simulink model "SensorlessHandoverTest"  (R2026b)
settings: Solver=FixedStepDiscrete  StopTime=handoverTestCfg.Duration  FixedStep=handoverCfg.Ts
PostLoadFcn:
  | addpath(fullfile(fileparts(get_param(bdroot,'FileName')),'..','build_process'));initialize_handover_test(bdroot);
model workspace (MAT data in the model file):
  handoverCfg.Ts = 5e-05
  handoverCfg.MinOmega = 100
  handoverCfg.MaxSpeedGap = 80
  handoverCfg.MaxPhaseGap = 0.9
  handoverCfg.MaxResidual = 1.5
  handoverCfg.CaptureTime = 0.01
  handoverCfg.BlendTime = 0.1
  handoverCfg.LossTime = 0.001
  handoverCfg.MaxPhaseInnovation = 0.15
  handoverCfg.AllowFlying = 1
  handoverCfg.Samples = [200; 2000; 20]
  handoverCfg.Vector = [5e-05; 100; 80; 0.9; 1.5; 200; 2000; 20; 0.15; 1]
  handoverCfg.State0 = [0; 0; 0; 0; 0; 0; 0; 0; 0]
  handoverTestCfg.Duration = 0.35
  handoverTestCfg.ElectricalSpeed = 200
  handoverTestCfg.InitialAngle = 0
  handoverTestCfg.StartupAngleOffset = 0.4
  handoverTestCfg.Ready = 1
  handoverTestCfg.StartupMode = 4
  handoverTestCfg.StartupFault = 0
  handoverTestCfg.ObserverValidTime = 0.02
  handoverTestCfg.ResidualNorm = 0.1
  handoverTestCfg.Enable = 1
  handoverTestCfg.Reset = 0
  testStim.time = [0 5e-05 0.0001 0.00015 0.0002 0.00025 0.0003 0.00035 0.0004 0.00045 0.0005 0.00055 ... (7001 elements, 7001x1)]
  testStim.signals.values = [0.4 0.41 0.42 0.43 0.44 0.45 0.46 0.47 0.48 0.49 0.5 0.51 ... (77011 elements, 7001x11)]
  testStim.signals.dimensions = 11
libraries: SensorlessHandover x1
settings Model: Creator=24322  LastModifiedBy=24322

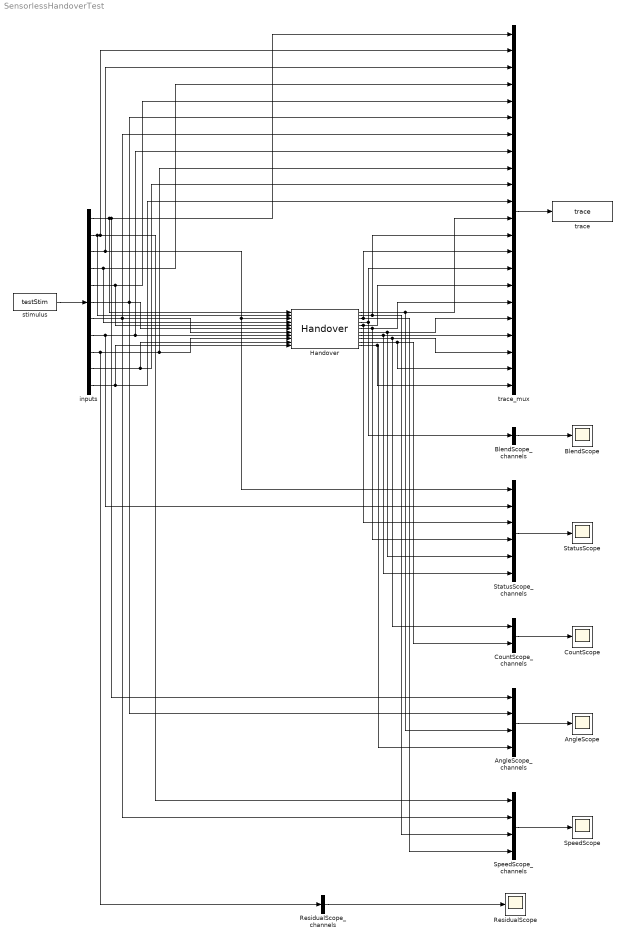
== system SensorlessHandoverTest ==
  AngleScope : Scope
  AngleScope_channels : Mux
  BlendScope : Scope
  BlendScope_channels : Mux  Inputs=1
  CountScope : Scope
  CountScope_channels : Mux  Inputs=2
  Handover : SensorlessHandover/Handover  handoverCfg=handoverCfg
  ResidualScope : Scope
  ResidualScope_channels : Mux  Inputs=1
  SpeedScope : Scope
  SpeedScope_channels : Mux
  StatusScope : Scope
  StatusScope_channels : Mux  Inputs=6
  inputs : Demux  Outputs=11
  stimulus : FromWorkspace  VariableName=testStim  SampleTime=handoverCfg.Ts  Interpolate=off  OutputAfterFinalValue=Holding final value
  trace : ToWorkspace  VariableName=trace  SaveFormat=Structure With Time  SampleTime=-1
  trace_mux : Mux  Inputs=22
  wires:
  ResidualScope_channels/1 -> ResidualScope/1
  CountScope_channels/1 -> CountScope/1
  StatusScope_channels/1 -> StatusScope/1
  BlendScope_channels/1 -> BlendScope/1
  SpeedScope_channels/1 -> SpeedScope/1
  AngleScope_channels/1 -> AngleScope/1
  Handover/11 -> trace_mux/22, AngleScope_channels/4
  Handover/10 -> trace_mux/21, CountScope_channels/2
  Handover/9 -> trace_mux/20, CountScope_channels/1
  Handover/8 -> trace_mux/19, StatusScope_channels/6
  Handover/7 -> trace_mux/18, StatusScope_channels/5
  Handover/6 -> trace_mux/17, StatusScope_channels/4
  Handover/5 -> trace_mux/16, StatusScope_channels/3
  Handover/4 -> trace_mux/15, BlendScope_channels/1
  Handover/3 -> trace_mux/14, SpeedScope_channels/4
  Handover/2 -> trace_mux/13, SpeedScope_channels/3
  Handover/1 -> trace_mux/12, AngleScope_channels/3
  inputs/11 -> Handover/11, trace_mux/11
  inputs/10 -> Handover/10, trace_mux/10
  inputs/9 -> Handover/9, trace_mux/9, ResidualScope_channels/1
  inputs/8 -> Handover/8, trace_mux/8, StatusScope_channels/2
  inputs/7 -> Handover/7, trace_mux/7, SpeedScope_channels/2
  inputs/6 -> Handover/6, trace_mux/6, AngleScope_channels/2
  inputs/5 -> Handover/5, trace_mux/5
  inputs/4 -> Handover/4, trace_mux/4
  inputs/3 -> Handover/3, StatusScope_channels/1, trace_mux/3
  inputs/2 -> trace_mux/2, SpeedScope_channels/1, Handover/2
  inputs/1 -> trace_mux/1, AngleScope_channels/1, Handover/1
  trace_mux/1 -> trace/1
  stimulus/1 -> inputs/1
